simulink model "FMT_DataSIM"  (R2026b)
settings: Solver=FixedStepDiscrete  StopTime=26  FixedStep=0.0005
undefined symbols (not defined in the file): fmt_flight_nav_width, SensorModelParameters, SensorTimingParameters
settings Model: DataDictionary=Flight_Parameters.sldd  Creator=26718  LastModifiedBy=26718
settings DataIOCC: ExternalInput=fmt_default_input('FMT_DataSIM')  LoadExternalInput=on
settings DebuggingCC: AlgebraicLoopMsg=error

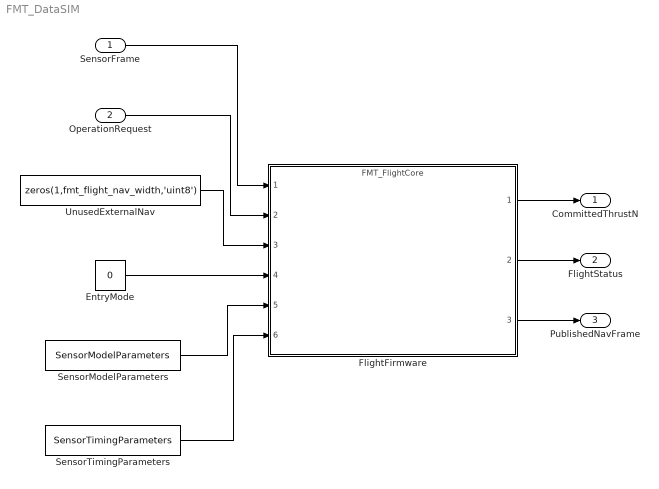
== system FMT_DataSIM ==
  SensorFrame : Inport  OutDataTypeStr=double  PortDimensions=18  SampleTime=0.0005  Interpolate=off
  OperationRequest : Inport  Port=2  OutDataTypeStr=double  PortDimensions=2  SampleTime=0.0005  Interpolate=off
  EntryMode : Constant  Value=0
  FlightFirmware : ModelReference  ModelNameDialog=FMT_FlightCore  SimulationMode=Normal  ModelReferenceVersion=1.1
  SensorModelParameters : Constant  Value=SensorModelParameters
  SensorTimingParameters : Constant  Value=SensorTimingParameters
  UnusedExternalNav : Constant  Value=zeros(1,fmt_flight_nav_width,'uint8')  OutDataTypeStr=uint8
  CommittedThrustN : Outport
  FlightStatus : Outport  Port=2
  PublishedNavFrame : Outport  Port=3
  wires:
  SensorTimingParameters/1 -> FlightFirmware/6
  SensorModelParameters/1 -> FlightFirmware/5
  OperationRequest/1 -> FlightFirmware/2
  UnusedExternalNav/1 -> FlightFirmware/3
  SensorFrame/1 -> FlightFirmware/1
  FlightFirmware/3 -> PublishedNavFrame/1
  FlightFirmware/2 -> FlightStatus/1
  FlightFirmware/1 -> CommittedThrustN/1
  EntryMode/1 -> FlightFirmware/4
